simulink model "self_balancing_robot_lqr_perfect_state"  (R2026b)
settings: Solver=VariableStepAuto
values from neighbouring files (symbols this model uses):
  A_ss = [0 1 0 0 ... (first row only)    [robot_params.m]
  Ad = sys_d.A    [robot_params.m]
  alpha_comp = 0.98    [robot_params.m]
  B_ss = [0 ... (first row only)    [robot_params.m]
  Bd = sys_d.B    [robot_params.m]
  C_meas = [1 0 0 0 ... (first row only)    [robot_params.m]    (also in version3_analysis.m)
  C_ss = eye(4)    [robot_params.m]
  D_ss = zeros(4,1)    [robot_params.m]
  disturbance_end = 4.1    [compare_pid_lqr.m]    (also in compare_v3.m = distEnd_list(i); version3_analysis.m = 5.1)
  disturbance_mag = 0.5    [compare_pid_lqr.m]    (also in compare_v3.m = distMag_list(i); version3_analysis.m = 0)
  disturbance_start = 4    [compare_pid_lqr.m]    (also in compare_v3.m = distStart_list(i); version3_analysis.m)
  gyro_bias = deg2rad(0.1)    [robot_params.m]
  K_lqr = K_lqr_nominal    [robot_params.m]
  sigma_gyro = deg2rad(0.5)    [robot_params.m]
  sigma_theta = deg2rad(0.2)    [robot_params.m]
  sigma_x = 0.002    [robot_params.m]
  theta0 = theta0_list(i)    [compare_v3.m]    (also in version3_analysis.m = deg2rad(5))
  Ts_sensor = 0.01    [robot_params.m]
undefined symbols (not defined in the file or in its folder): L_kf
settings Model: Creator=legne  LastModifiedBy=legne

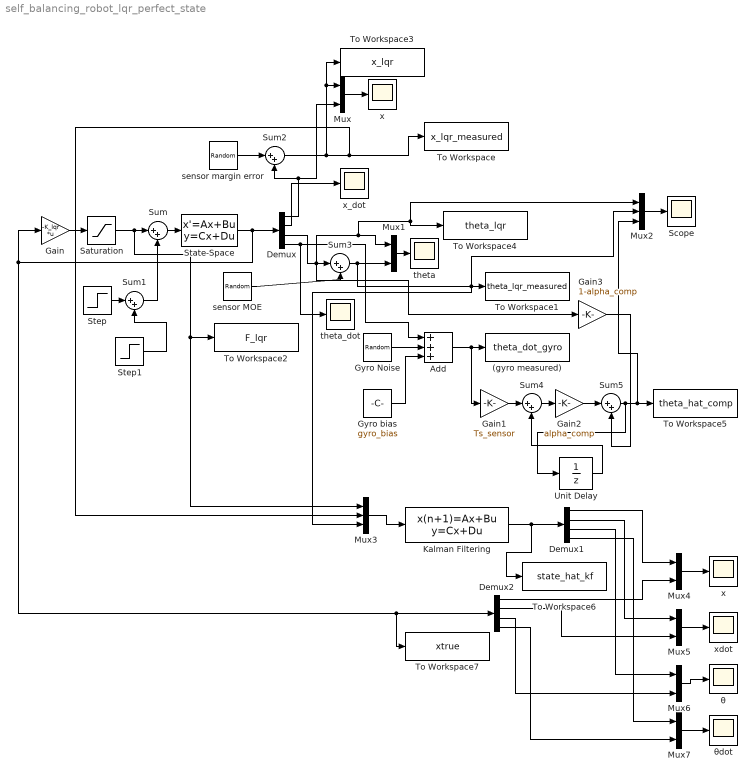
== system self_balancing_robot_lqr_perfect_state ==
  " x" : Scope
      settings: ActiveDisplayYMinimum=-0.030209826975059272  ActiveDisplayYMaximum=0.13907253479299955  DataLoggingVariableName=ScopeData10
  " xdot" : Scope
      settings: DataLoggingVariableName=ScopeData5
  (gyro measured) : ToWorkspace  VariableName=theta_dot_gyro  SaveFormat=Timeseries  SampleTime=-1
  Add : Sum  Inputs=+++
  Demux : Demux
  Demux1 : Demux
  Demux2 : Demux
  Gain : Gain  Gain=-K_lqr  Multiplication=Matrix(K*u)
  Gain1 : Gain  Gain=Ts_sensor
  Gain2 : Gain  Gain=alpha_comp
  Gain3 : Gain  Gain=1-alpha_comp
  Gyro Noise : RandomNumber  Variance=sigma_gyro^2  SampleTime=Ts_sensor
  Gyro bias : Constant  Value=gyro_bias
  Kalman Filtering : DiscreteStateSpace  A=Ad - L_kf*C_meas  B=[Bd L_kf]  C=eye(4)  D=zeros(4,3)  InitialCondition=[0; 0; theta0; 0]  SampleTime=Ts_sensor
  Mux{,1,4..7} (6 alike) : Mux  Inputs=2
  Mux2 : Mux  Inputs=3
  Mux3 : Mux  Inputs=3
  Saturation : Saturate  UpperLimit=2  LowerLimit=-2
  Scope : Scope
      settings: ActiveDisplayYMinimum=-1.9857185551710963  ActiveDisplayYMaximum=1.2557966677909767  DataLoggingVariableName=ScopeData4
  State-Space : StateSpace  A=A_ss  B=B_ss  C=C_ss  D=D_ss  InitialCondition=[0;0;0.0873;0]
  Step : Step  Time=disturbance_start  FinalValue=disturbance_mag  SampleTime=0
  Step1 : Step  Time=disturbance_end  FinalValue=-disturbance_mag  SampleTime=0
  Sum{,1..5} (6 alike) : Sum  Inputs=|++
  To Workspace : ToWorkspace  VariableName=x_lqr_measured  SaveFormat=Timeseries  SampleTime=-1
  To Workspace1 : ToWorkspace  VariableName=theta_lqr_measured  SaveFormat=Timeseries  SampleTime=-1
  To Workspace2 : ToWorkspace  VariableName=F_lqr  SaveFormat=Timeseries  SampleTime=-1
  To Workspace3 : ToWorkspace  VariableName=x_lqr  SaveFormat=Timeseries  SampleTime=-1
  To Workspace4 : ToWorkspace  VariableName=theta_lqr  SaveFormat=Timeseries  SampleTime=-1
  To Workspace5 : ToWorkspace  VariableName=theta_hat_comp  SaveFormat=Timeseries  SampleTime=-1
  To Workspace6 : ToWorkspace  VariableName=state_hat_kf  SaveFormat=Timeseries  SampleTime=-1
  To Workspace7 : ToWorkspace  VariableName=xtrue  SaveFormat=Timeseries  SampleTime=-1
  Unit Delay : UnitDelay  InitialCondition=theta0  SampleTime=Ts_sensor
  sensor MOE : RandomNumber  Variance=sigma_theta^2  SampleTime=Ts_sensor
  sensor margin error : RandomNumber  Variance=sigma_x^2  SampleTime=Ts_sensor
  theta : Scope
      settings: ActiveDisplayYMinimum=-0.049162029343614896  ActiveDisplayYMaximum=0.10698073090282449  DataLoggingVariableName=ScopeData2
  theta_dot : Scope
      settings: DataLoggingVariableName=ScopeData3
  x : Scope
      settings: ActiveDisplayYMinimum=-0.045234276165425649  ActiveDisplayYMaximum=0.18750966519906606
  x_dot : Scope
      settings: ActiveDisplayYMinimum=-0.12450705891050609  ActiveDisplayYMaximum=0.29480089468753706
  θ : Scope
      settings: ActiveDisplayYMinimum=-0.044224865334267449  ActiveDisplayYMaximum=0.10297694496662257  DataLoggingVariableName=ScopeData11
  θdot : Scope
      settings: DataLoggingVariableName=ScopeData12
  wires:
  State-Space/1 -> To Workspace7/1, Demux2/1, Gain/1, Demux/1
  Demux/2 -> x_dot/1
  Demux/4 -> theta_dot/1, Add/1
  Gain/1 -> Saturation/1
  Saturation/1 -> Mux3/1, To Workspace2/1, Sum/1
  Sum/1 -> State-Space/1
  Step/1 -> Sum1/1
  Step1/1 -> Sum1/2
  Sum1/1 -> Sum/2
  Demux/1 -> To Workspace3/1, Mux/1, Sum2/2
  sensor margin error/1 -> Sum2/1
  Sum2/1 -> Mux/2, Mux3/2, To Workspace/1
  Demux/3 -> Mux2/1, To Workspace4/1, Mux1/1, Sum3/1, Gain3/1
  Sum3/1 -> Mux3/3, To Workspace1/1, Mux2/2, Mux1/2
  sensor MOE/1 -> Sum3/2
  Mux/1 -> x/1
  Mux1/1 -> theta/1
  Gyro bias/1 -> Add/3
  Gyro Noise/1 -> Add/2
  Add/1 -> Gain1/1, (gyro measured)/1
  Gain1/1 -> Sum4/1
  Sum4/1 -> Gain2/1
  Gain2/1 -> Sum5/1
  Sum5/1 -> Unit Delay/1, Mux2/3, To Workspace5/1
  Gain3/1 -> Sum5/2
  Unit Delay/1 -> Sum4/2
  Mux2/1 -> Scope/1
  Mux3/1 -> Kalman Filtering/1
  Kalman Filtering/1 -> To Workspace6/1, Demux1/1
  Demux1/1 -> Mux4/1
  Demux2/1 -> Mux4/2
  Demux1/2 -> Mux5/1
  Demux2/2 -> Mux5/2
  Demux2/4 -> Mux7/2
  Demux1/3 -> Mux6/1
  Demux2/3 -> Mux6/2
  Demux1/4 -> Mux7/1
  Mux4/1 -> " x"/1
  Mux5/1 -> " xdot"/1
  Mux6/1 -> θ/1
  Mux7/1 -> θdot/1
